simulink model "sm_car"  (R2025a)
settings: Solver=ode23t  StartTime=0.0  StopTime=400  MaxStep=0.4  RelTol=1e-3  AbsTol=1e-3  EnableMultiTasking=on
PreLoadFcn:
  | % Due to usability issue in Repeating Sequence block
  | warning('off','Simulink:Masking:Invalid');
  | 
  | % Eliminate unnecessary warnings in inactive variants
  | % Warnings generated only if you click through inactive variant
  | warning('off','MATLAB:nonExistentField');
  | warning('off','Simulink:Parameters:BlkParamUndefined');
PostLoadFcn:
  | set_param([bdroot '/Vehicle'],'popup_trailer','Off')
  | warning('off','sm:sli:setup:compile:LocalSolverNotSupported')
  | %sm_car_config_maneuver(bdroot,'WOT Braking');
  | sm_car_config_vehicle(bdroot,'false');
  | sm_car_config_logging(bdroot);
InitFcn:
  | sm_car_config_camera;
  | Vehicle = sm_car_vehcfg_checkConfig(Vehicle);
  | sm_car_check_tire_model(bdroot);
StartFcn:
  | tic;
StopFcn:
  | Elapsed_Sim_Time = toc;
  | % disp(['Elapsed Sim Time = ' num2str(Elapsed_Sim_Time)]);
undefined symbols (not defined in the file): Axle1D, AxleIn, Camera, Control, Driver, Free, Init, Maneuver, Pedal, RaceFix, RaceSpin, Scene, ShaftL1, ShaftL2, ShaftR1, ShaftR2, Soft, Stiff, Visual, X, xy_data_car_side, Y, Z
libraries: sm_lib x1546, nesl_utility x528, fl_lib x480, SimscapeFluids_lib x61, sdl_lib x49, simulink x29, ee_lib x7, simulink_extras x6, Linkage_Systems x4, Tire_1x2x x4, AntiRollBar_Systems x2, Linkage_Decoupled x2
(part 8 of 79)

== system sm_car/Vehicle/Vehicle/Chassis/Body ==
  Body Geometry : Subsystem  Variant=on  VariantControlMode=label  VariantControl=Variant1  LabelModeActiveChoice=CAD_FSAE_Achilles  mask(Variants for Vehicle Body Geometry){BodyGeometry=BodyGeometry, VariantLabel=BodyGeometry.class.Value}
      mask prompts: VariantLabel "Variant Label"
      mask help: Select option and provide parameters for vehicle body geometry. Option is chosen by string provided in Variant Label. The parameters for the selected option is contained in Body Geometry data structure.
      mask init:
      | curblk = gcb;
      | 
      | % Set variant for this block 
      | set_param(curblk,'LabelModeActiveChoice',VariantLabel);
      settings: AttributesFormatString=%<LabelModeActiveChoice>
  Body Load : Subsystem  Variant=on  VariantControlMode=label  VariantControl=Variant1  LabelModeActiveChoice=None  mask(Variants for Vehicle Body Load){BodyLoad=BodyLoad, VariantLabel=BodyLoad.class.Value}
      mask prompts: VariantLabel "Variant Label"
      mask help: Select option and provide parameters for vehicle body load. Option is chosen by string provided in Variant Label. The parameters for the selected option is contained in Body Load data structure.
      mask init:
      | curblk = gcb;
      | 
      | % Set variant for this block 
      | set_param(curblk,'LabelModeActiveChoice',VariantLabel);
      settings: AttributesFormatString=%<LabelModeActiveChoice>
  Body Mass and Inertia : sm_lib/Body Elements/Spherical Solid  SphereRadius=size_chassis_hp_cg  SphereRadiusUnits=m  ExportEntireGeometry=off  InertiaType=Custom  BasedOnType=Density  Density=312*0.6  DensityUnits=kg/m^3  Mass=chassis_mass  MassUnits=kg  CenterOfMass=[0 0 0]  CenterOfMassUnits=m  MomentsOfInertia=chassis_inertia  MomentsOfInertiaUnits=kg*m^2  ProductsOfInertia=[0 0 0]  ProductsOfInertiaUnits=kg*m^2  GraphicType=FromGeometry  MarkerShape=Sphere  MarkerSize=10  GraphicVisPropType=SimpleVisualProperties  GraphicDiffuseColor=clr_chassis_hp_cg  GraphicOpacity=opc_chassis_hp_cg  GraphicSpecularColor=[0.5 0.5 0.5 1.0]  GraphicAmbientColor=[0.15 0.15 0.15 1.0]  GraphicEmissiveColor=[0.0 0.0 0.0 1.0]  GraphicShininess=75  DoExposeReferenceFrame=on  SerializedFrames=<Frames/>
  Body Sensor : Subsystem  mask{offset_body_sensor=[0 0 0]}
      mask prompts: offset_body_sensor "Sensor Frame Offset [x y z] (m)"
  Bus Creator : BusCreator  Inputs=4
  Passenger FL : Subsystem  Variant=on  VariantControlMode=label  LabelModeActiveChoice=None  mask{Passenger=Passenger.FL, VariantLabel=Passenger.FL.class.Value}
      mask prompts: Passenger "Passenger Data"; VariantLabel "Variant Label"
      mask init:
      | curblk = gcb;
      | 
      | % Set variant for this block 
      | set_param(curblk,'LabelModeActiveChoice',VariantLabel);
      settings: AttributesFormatString=%<LabelModeActiveChoice>
  Passenger FR : Subsystem  Variant=on  VariantControlMode=label  LabelModeActiveChoice=None  mask{Passenger=Passenger.FR, VariantLabel=Passenger.FR.class.Value}
      mask prompts: Passenger "Passenger Data"; VariantLabel "Variant Label"
      mask init:
      | curblk = gcb;
      | 
      | % Set variant for this block 
      | set_param(curblk,'LabelModeActiveChoice',VariantLabel);
      settings: AttributesFormatString=%<LabelModeActiveChoice>
  Passenger RL : Subsystem  Variant=on  VariantControlMode=label  LabelModeActiveChoice=None  mask{Passenger=Passenger.RL, VariantLabel=Passenger.RL.class.Value}
      mask prompts: Passenger "Passenger Data"; VariantLabel "Variant Label"
      mask init:
      | curblk = gcb;
      | 
      | % Set variant for this block 
      | set_param(curblk,'LabelModeActiveChoice',VariantLabel);
      settings: AttributesFormatString=%<LabelModeActiveChoice>
  Passenger RR : Subsystem  Variant=on  VariantControlMode=label  LabelModeActiveChoice=None  mask{Passenger=Passenger.RR, VariantLabel=Passenger.RR.class.Value}
      mask prompts: Passenger "Passenger Data"; VariantLabel "Variant Label"
      mask init:
      | curblk = gcb;
      | 
      | % Set variant for this block 
      | set_param(curblk,'LabelModeActiveChoice',VariantLabel);
      settings: AttributesFormatString=%<LabelModeActiveChoice>
  Reference Frame Front Hitch : sm_lib/Frames and Transforms/Reference Frame
  Reference Frame Rear Hitch : sm_lib/Frames and Transforms/Reference Frame
  Transform Body CG : sm_lib/Frames and Transforms/Rigid Transform  RotationMethod=None  FollAlignAxisA=+X  BaseAlignAxisA=+Y  FollAlignAxisB=+Y  BaseAlignAxisB=+Z  RotationStandardAxis=+Z  RotationAngle=0.0  RotationAngleUnits=deg  RotationArbitraryAxis=[0 0 1]  RotationSequenceAxes=FollowerAxes  RotationSequence=XYX  RotationSequenceAngles=[0 0 0]  RotationSequenceAnglesUnits=deg  RotationMatrix=[1 0 0; 0 1 0; 0 0 1]  Quaternion=[1 0 0 0]  TranslationMethod=Cartesian  TranslationCartesianOffset=hp_chassis_cg  TranslationCartesianOffsetUnits=m  TranslationStandardAxis=+Z  TranslationStandardOffset=0  TranslationStandardOffsetUnits=m  TranslationROffset=0  TranslationROffsetUnits=m  TranslationThetaOffset=0  TranslationThetaOffsetUnits=deg  TranslationZOffset=0  TranslationZOffsetUnits=m
  Transform Front Hitch : sm_lib/Frames and Transforms/Rigid Transform  RotationMethod=None  FollAlignAxisA=+X  BaseAlignAxisA=+Y  FollAlignAxisB=+Y  BaseAlignAxisB=+Z  RotationStandardAxis=+Z  RotationAngle=0.0  RotationAngleUnits=deg  RotationArbitraryAxis=[0 0 1]  RotationSequenceAxes=FollowerAxes  RotationSequence=XYX  RotationSequenceAngles=[0 0 0]  RotationSequenceAnglesUnits=deg  RotationMatrix=[1 0 0; 0 1 0; 0 0 1]  Quaternion=[1 0 0 0]  TranslationMethod=Cartesian  TranslationCartesianOffset=hp_mount_hitchf  TranslationCartesianOffsetUnits=m  TranslationStandardAxis=-X  TranslationStandardOffset=0  TranslationStandardOffsetUnits=m  TranslationROffset=0  TranslationROffsetUnits=m  TranslationThetaOffset=0  TranslationThetaOffsetUnits=deg  TranslationZOffset=0  TranslationZOffsetUnits=m
  Transform Mount A1 : sm_lib/Frames and Transforms/Rigid Transform  RotationMethod=None  FollAlignAxisA=+X  BaseAlignAxisA=+Y  FollAlignAxisB=+Y  BaseAlignAxisB=+Z  RotationStandardAxis=+Z  RotationAngle=0.0  RotationAngleUnits=deg  RotationArbitraryAxis=[0 0 1]  RotationSequenceAxes=FollowerAxes  RotationSequence=XYX  RotationSequenceAngles=[0 0 0]  RotationSequenceAnglesUnits=deg  RotationMatrix=[1 0 0; 0 1 0; 0 0 1]  Quaternion=[1 0 0 0]  TranslationMethod=Cartesian  TranslationCartesianOffset=hp_mount_a1  TranslationCartesianOffsetUnits=m  TranslationStandardAxis=+X  TranslationStandardOffset=0  TranslationStandardOffsetUnits=m  TranslationROffset=0  TranslationROffsetUnits=m  TranslationThetaOffset=0  TranslationThetaOffsetUnits=deg  TranslationZOffset=0  TranslationZOffsetUnits=m
  Transform Mount A2 : sm_lib/Frames and Transforms/Rigid Transform  RotationMethod=None  FollAlignAxisA=+X  BaseAlignAxisA=+Y  FollAlignAxisB=+Y  BaseAlignAxisB=+Z  RotationStandardAxis=+Z  RotationAngle=0.0  RotationAngleUnits=deg  RotationArbitraryAxis=[0 0 1]  RotationSequenceAxes=FollowerAxes  RotationSequence=XYX  RotationSequenceAngles=[0 0 0]  RotationSequenceAnglesUnits=deg  RotationMatrix=[1 0 0; 0 1 0; 0 0 1]  Quaternion=[1 0 0 0]  TranslationMethod=Cartesian  TranslationCartesianOffset=hp_mount_a2  TranslationCartesianOffsetUnits=m  TranslationStandardAxis=-X  TranslationStandardOffset=0  TranslationStandardOffsetUnits=m  TranslationROffset=0  TranslationROffsetUnits=m  TranslationThetaOffset=0  TranslationThetaOffsetUnits=deg  TranslationZOffset=0  TranslationZOffsetUnits=m
  Transform Power Mount : sm_lib/Frames and Transforms/Rigid Transform  RotationMethod=None  FollAlignAxisA=+X  BaseAlignAxisA=+Y  FollAlignAxisB=+Y  BaseAlignAxisB=+Z  RotationStandardAxis=+Z  RotationAngle=0.0  RotationAngleUnits=deg  RotationArbitraryAxis=[0 0 1]  RotationSequenceAxes=FollowerAxes  RotationSequence=XYX  RotationSequenceAngles=[0 0 0]  RotationSequenceAnglesUnits=deg  RotationMatrix=[1 0 0; 0 1 0; 0 0 1]  Quaternion=[1 0 0 0]  TranslationMethod=Cartesian  TranslationCartesianOffset=hp_mount_power  TranslationCartesianOffsetUnits=m  TranslationStandardAxis=+Z  TranslationStandardOffset=0  TranslationStandardOffsetUnits=m  TranslationROffset=0  TranslationROffsetUnits=m  TranslationThetaOffset=0  TranslationThetaOffsetUnits=deg  TranslationZOffset=0  TranslationZOffsetUnits=m
  Transform Rear Hitch : sm_lib/Frames and Transforms/Rigid Transform  RotationMethod=None  FollAlignAxisA=+X  BaseAlignAxisA=+Y  FollAlignAxisB=+Y  BaseAlignAxisB=+Z  RotationStandardAxis=+Z  RotationAngle=0.0  RotationAngleUnits=deg  RotationArbitraryAxis=[0 0 1]  RotationSequenceAxes=FollowerAxes  RotationSequence=XYX  RotationSequenceAngles=[0 0 0]  RotationSequenceAnglesUnits=deg  RotationMatrix=[1 0 0; 0 1 0; 0 0 1]  Quaternion=[1 0 0 0]  TranslationMethod=Cartesian  TranslationCartesianOffset=hp_mount_hitchr  TranslationCartesianOffsetUnits=m  TranslationStandardAxis=-X  TranslationStandardOffset=0  TranslationStandardOffsetUnits=m  TranslationROffset=0  TranslationROffsetUnits=m  TranslationThetaOffset=0  TranslationThetaOffsetUnits=deg  TranslationZOffset=0  TranslationZOffsetUnits=m
  Vis HP Mount A1 : sm_lib/Body Elements/Spherical Solid  SphereRadius=size_chassis_hp_cg  SphereRadiusUnits=m  ExportEntireGeometry=off  InertiaType=PointMass  BasedOnType=Density  Density=312*0.6  DensityUnits=kg/m^3  Mass=0  MassUnits=kg  CenterOfMass=[0 0 0]  CenterOfMassUnits=m  MomentsOfInertia=[1 1 1]  MomentsOfInertiaUnits=kg*m^2  ProductsOfInertia=[0 0 0]  ProductsOfInertiaUnits=kg*m^2  GraphicType=FromGeometry  MarkerShape=Sphere  MarkerSize=10  GraphicVisPropType=SimpleVisualProperties  GraphicDiffuseColor=clr_chassis_hp_cg  GraphicOpacity=opc_chassis_hp_cg  GraphicSpecularColor=[0.5 0.5 0.5 1.0]  GraphicAmbientColor=[0.15 0.15 0.15 1.0]  GraphicEmissiveColor=[0.0 0.0 0.0 1.0]  GraphicShininess=75  DoExposeReferenceFrame=on  SerializedFrames=<Frames/>
  Vis HP Mount A2 : sm_lib/Body Elements/Spherical Solid  SphereRadius=size_chassis_hp_cg  SphereRadiusUnits=m  ExportEntireGeometry=off  InertiaType=PointMass  BasedOnType=Density  Density=312*0.6  DensityUnits=kg/m^3  Mass=0  MassUnits=kg  CenterOfMass=[0 0 0]  CenterOfMassUnits=m  MomentsOfInertia=[1 1 1]  MomentsOfInertiaUnits=kg*m^2  ProductsOfInertia=[0 0 0]  ProductsOfInertiaUnits=kg*m^2  GraphicType=FromGeometry  MarkerShape=Sphere  MarkerSize=10  GraphicVisPropType=SimpleVisualProperties  GraphicDiffuseColor=clr_chassis_hp_cg  GraphicOpacity=opc_chassis_hp_cg  GraphicSpecularColor=[0.5 0.5 0.5 1.0]  GraphicAmbientColor=[0.15 0.15 0.15 1.0]  GraphicEmissiveColor=[0.0 0.0 0.0 1.0]  GraphicShininess=75  DoExposeReferenceFrame=on  SerializedFrames=<Frames/>
  HF : PMIOPort  Side=Left
  A1 : PMIOPort  Port=2  Side=Right
  Pwr : PMIOPort  Port=3  Side=Left
  W : PMIOPort  Port=4  Side=Left
  A2 : PMIOPort  Port=5  Side=Right
  HR : PMIOPort  Port=6  Side=Left
  Out Bus Element : Outport  VectorParamsAs1DForOutWhenUnconnected=off  PortName=m  Element=Passengers
  Out Bus Element1 : Outport  VectorParamsAs1DForOutWhenUnconnected=off  PortName=m  Element=CG
  wires:
  Body Sensor/1(Body) -> Out Bus Element1/1
  [PassRR] -> Bus Creator/4  "RR"
  [PassRL] -> Bus Creator/3  "RL"
  Passenger RR/1(m) -> [PassRR]
  Passenger RL/1(m) -> [PassRL]
  Passenger FL/1(m) -> [PassFL]
  [PassFR] -> Bus Creator/2  "FR"
  [PassFL] -> Bus Creator/1  "FL"
  Passenger FR/1(m) -> [PassFR]
  Bus Creator/1 -> Out Bus Element/1
  connections:
  Passenger RR/LConn1 -- Passenger FR/LConn1 -- Passenger FL/LConn1 -- Body Geometry/LConn1 -- Passenger RL/LConn1
  Reference Frame Front Hitch/RConn1 -- Transform Front Hitch/RConn1 -- HF/RConn1
  Reference Frame Rear Hitch/RConn1 -- Transform Rear Hitch/RConn1 -- HR/RConn1
  Pwr/RConn1 -- Transform Power Mount/RConn1
  Transform Mount A2/RConn1 -- Vis HP Mount A2/RConn1 -- A2/RConn1
  Transform Mount A1/RConn1 -- Body Load/LConn1 -- Body Geometry/RConn1 -- A1/RConn1 -- Vis HP Mount A1/RConn1
  Transform Body CG/RConn1 -- Body Sensor/LConn1 -- Body Mass and Inertia/RConn1
  W/RConn1 -- Transform Rear Hitch/LConn1 -- Transform Front Hitch/LConn1 -- Transform Mount A1/LConn1 -- Transform Mount A2/LConn1 -- Transform Power Mount/LConn1 -- Transform Body CG/LConn1

== system sm_car/Vehicle/Vehicle/Chassis/Damper ==
  "Ctrl " : Inport
  Decoupled : Subsystem  VariantControl=Decoupled  mask(Roll and Heave Dampers){}
      mask help: Models dampers in a suspension design that decouples damping for body roll and heave .
  Independent : Subsystem  VariantControl=Independent  mask(Independent Dampers){}
      mask help: Models independent left and right dampers on two axles
  " L1" : PMIOPort  Side=Left
  " R1" : PMIOPort  Port=2  Side=Right
  " L2" : PMIOPort  Port=3  Side=Left
  " R2" : PMIOPort  Port=4  Side=Right
  " meas" : Outport  VectorParamsAs1DForOutWhenUnconnected=off

== system sm_car/Vehicle/Vehicle/Chassis/Spring ==
  "Ctrl " : Inport
  Decoupled : Subsystem  VariantControl=Decoupled  mask(Roll and Heave Springs){}
      mask help: Models springs in a suspension design that decouples stiffness for body roll and heave .
  Independent : Subsystem  VariantControl=Independent  mask(Independent Springs){}
      mask help: Models independent left and right springs on two axles
  " L1" : PMIOPort  Side=Left
  R1 : PMIOPort  Port=2  Side=Right
  " L2" : PMIOPort  Port=3  Side=Left
  R2 : PMIOPort  Port=4  Side=Right
  " meas" : Outport  VectorParamsAs1DForOutWhenUnconnected=off

== system sm_car/Vehicle/Vehicle/Chassis/SuspA1 ==
  "CtrlBus " : Inport
  DrvBus : Inport  Port=2
  Linkage : Subsystem  VariantControl=Linkage  mask(Linkage Suspension){}
      mask help: Models suspension using linkages, including double-wishbone and multi-link suspensions. This subsystem models the suspension, spring and damper parts, and optional steering system. The displacement of the springs and dampers are modeled here and the forces are modeled in a separate subsystem.
      mask Display: image('sm_car_vehicle_susp_linkage_IMAGE.png');
  Linkage Decoupled : Subsystem  VariantControl=Decoupled  mask(Linkage Decoupled){}
      mask help: Models suspension using a linkage where the stiffness and damping for the roll and heave degrees of freedom are decoupled. Includes suspension, spring and damper parts, and optional steering system. The displacement of the springs and dampers are modeled here and the forces are modeled in a separate subsystem.
      mask Display: image('sm_car_vehicle_susp_linkage_decouple_IMAGE.png');
  WCL : PMIOPort  Side=Left
  Ref : PMIOPort  Port=2  Side=Right
  WCR : PMIOPort  Port=3  Side=Right
  AxleL : PMIOPort  Port=4  Side=Left
  AxleR : PMIOPort  Port=5  Side=Right
  SprL : PMIOPort  Port=6  Side=Left
  SprR : PMIOPort  Port=7  Side=Right
  DmpL : PMIOPort  Port=8  Side=Left
  DmpR : PMIOPort  Port=9  Side=Right
  OutBus : Outport  VectorParamsAs1DForOutWhenUnconnected=off

== system sm_car/Vehicle/Vehicle/Chassis/SuspA2 ==
  "CtrlBus " : Inport
  DrvBus : Inport  Port=2
  Linkage : Subsystem  VariantControl=Linkage  mask(Linkage Suspension){}
      mask help: Models suspension using linkages, including double-wishbone and multi-link suspensions. This subsystem models the suspension, spring and damper parts, and optional steering system. The displacement of the springs and dampers are modeled here and the forces are modeled in a separate subsystem.
      mask Display: image('sm_car_vehicle_susp_linkage_IMAGE.png');
  Linkage Decoupled : Suspension_Linkage_Decoupled/Linkage Decoupled  VariantControl=Decoupled
  WCL : PMIOPort  Side=Left
  Ref : PMIOPort  Port=2  Side=Right
  WCR : PMIOPort  Port=3  Side=Right
  AxleL : PMIOPort  Port=4  Side=Left
  AxleR : PMIOPort  Port=5  Side=Right
  SprL : PMIOPort  Port=6  Side=Left
  SprR : PMIOPort  Port=7  Side=Right
  DmpL : PMIOPort  Port=8  Side=Left
  DmpR : PMIOPort  Port=9  Side=Right
  OutBus : Outport  VectorParamsAs1DForOutWhenUnconnected=off

== system sm_car/Vehicle/Vehicle/Powertrain/Driveline ==
  CtrlBus : Inport
  L1 R1 L2 R2 : Subsystem  Tag=PublishSubsystem  VariantControl=L1_R1_L2_R2  mask(Driveline, Two-Axle, Four Input Shaft){}
      mask help: Models two-axle driveline with four separate shafts. The shafts are connected independently to the wheels.
      mask Display: image('sm_car_vehicle_driveline_axle2_l1_r1_l2_r2_IMAGE.png');
  A1 : PMIOPort  Side=Left
  A2 : PMIOPort  Port=2  Side=Right
  L1 : PMIOPort  Port=3  Side=Left
  R1 : PMIOPort  Port=4  Side=Right
  L2 : PMIOPort  Port=5  Side=Left
  R2 : PMIOPort  Port=6  Side=Right
  Shafts : PMIOPort  Port=7  Side=Left
  " o" : PMIOPort  Port=8  Side=Right
  OutD : Outport  VectorParamsAs1DForOutWhenUnconnected=off

== system sm_car/Vehicle/Vehicle/Powertrain/Power ==
  CtrlBus : Inport
  VehBus : Inport  Port=2
  Electric L1 R1 L2 R2 : Subsystem  VariantControl=Electric_L1_R1_L2_R2  mask(Electric Propulsion with Four Motors){Power=Powertrain.Power}
      mask prompts: Power "Power 4 Motor (structure)"
      mask help: Four electric motors with optional cooling system. Physical connections for the four motor shafts are in bus Shafts.
      mask Display: image('sm_car_vehicle_power_e4motor_IMAGE.png');
  Shafts : PMIOPort  Side=Left
  Ref : PMIOPort  Port=2  Side=Right
  OutP : Outport  VectorParamsAs1DForOutWhenUnconnected=off

== system sm_car/Vehicle/Vehicle/Wheel Spin/Free ==
  note: For kinematics and compliance tests, the wheels need to be locked so they cannot spin.
      |
      | For all other tests, they should be free to rotate.
  L1 : PMIOPort  Side=Left
  L2 : PMIOPort  Port=2  Side=Left
  R1 : PMIOPort  Port=3  Side=Right
  R2 : PMIOPort  Port=4  Side=Right

== system sm_car/World/Scene/CRG Hockenheim/Finish Line ==
  L1 : Subsystem  mask{square_lwh=[0.01 1 1]}
      mask prompts: square_lwh "Size [l w h] (m)"
  L2 : Subsystem  mask{square_lwh=[0.01 1 1]}
      mask prompts: square_lwh "Size [l w h] (m)"
  L3 : Subsystem  mask{square_lwh=[0.01 1 1]}
      mask prompts: square_lwh "Size [l w h] (m)"
  L4 : Subsystem  mask{square_lwh=[0.01 1 1]}
      mask prompts: square_lwh "Size [l w h] (m)"
  L5 : Subsystem  mask{square_lwh=[0.01 1 1]}
      mask prompts: square_lwh "Size [l w h] (m)"
  Post L : sm_lib/Body Elements/Cylindrical Solid  CylinderRadius=post_r  CylinderRadiusUnits=m  CylinderLength=post_h  CylinderLengthUnits=m  ExportEntireGeometry=off  InertiaType=CalculateFromGeometry  BasedOnType=Density  Density=1000  DensityUnits=kg/m^3  Mass=1  MassUnits=kg  CenterOfMass=[0 0 0]  CenterOfMassUnits=m  MomentsOfInertia=[1 1 1]  MomentsOfInertiaUnits=kg*m^2  ProductsOfInertia=[0 0 0]  ProductsOfInertiaUnits=kg*m^2  GraphicType=FromGeometry  MarkerShape=Sphere  MarkerSize=10  GraphicVisPropType=SimpleVisualProperties  GraphicDiffuseColor=post_clr  GraphicOpacity=post_opc  GraphicSpecularColor=[0.5 0.5 0.5 1.0]  GraphicAmbientColor=[0.15 0.15 0.15 1.0]  GraphicEmissiveColor=[0.0 0.0 0.0 1.0]  GraphicShininess=75  DoExposeReferenceFrame=off  SerializedFrames=<Frames><Frame><Id>Frame1</Id><Value><Name>B</Name><Origin><Source>GeometricFeature</Source><FeatureName>bottom surface</FeatureName></Origin><PrimaryAxis><DefinedDirection>+Z</DefinedDirection><Source>ReferenceFrame</Source><SourceDirection>+Z</SourceDirection><FeatureName></FeatureName></PrimaryAxis><SecondaryAxis><DefinedDirection>+X</DefinedDirection><Source>ReferenceFrame</Source><SourceDirection>+X</SourceDirection><FeatureName></FeatureName></SecondaryAxis></Value></Frame><Frame><Id>Frame2</Id><Value><Name>T</Name><Origin><Source>GeometricFeature</Source><FeatureName>top surface</FeatureName></Origin><PrimaryAxis><DefinedDirection>+Z</DefinedDirection><Source>ReferenceFrame</Source><SourceDirection>+Z</SourceDirection><FeatureName></FeatureName></PrimaryAxis><SecondaryAxis><DefinedDirection>+X</DefinedDirection><Source>ReferenceFrame</Source><SourceDirection>+X</SourceDirection><FeatureName></FeatureName></SecondaryAxis></Value></Frame></Frames>
  Post R : sm_lib/Body Elements/Cylindrical Solid  CylinderRadius=post_r  CylinderRadiusUnits=m  CylinderLength=post_h  CylinderLengthUnits=m  ExportEntireGeometry=off  InertiaType=CalculateFromGeometry  BasedOnType=Density  Density=1000  DensityUnits=kg/m^3  Mass=1  MassUnits=kg  CenterOfMass=[0 0 0]  CenterOfMassUnits=m  MomentsOfInertia=[1 1 1]  MomentsOfInertiaUnits=kg*m^2  ProductsOfInertia=[0 0 0]  ProductsOfInertiaUnits=kg*m^2  GraphicType=FromGeometry  MarkerShape=Sphere  MarkerSize=10  GraphicVisPropType=SimpleVisualProperties  GraphicDiffuseColor=post_clr  GraphicOpacity=post_opc  GraphicSpecularColor=[0.5 0.5 0.5 1.0]  GraphicAmbientColor=[0.15 0.15 0.15 1.0]  GraphicEmissiveColor=[0.0 0.0 0.0 1.0]  GraphicShininess=75  DoExposeReferenceFrame=off  SerializedFrames=<Frames><Frame><Id>Frame1</Id><Value><Name>B</Name><Origin><Source>GeometricFeature</Source><FeatureName>bottom surface</FeatureName></Origin><PrimaryAxis><DefinedDirection>+Z</DefinedDirection><Source>ReferenceFrame</Source><SourceDirection>+Z</SourceDirection><FeatureName></FeatureName></PrimaryAxis><SecondaryAxis><DefinedDirection>+X</DefinedDirection><Source>ReferenceFrame</Source><SourceDirection>+X</SourceDirection><FeatureName></FeatureName></SecondaryAxis></Value></Frame><Frame><Id>Frame2</Id><Value><Name>T</Name><Origin><Source>GeometricFeature</Source><FeatureName>top surface</FeatureName></Origin><PrimaryAxis><DefinedDirection>+Z</DefinedDirection><Source>ReferenceFrame</Source><SourceDirection>+Z</SourceDirection><FeatureName></FeatureName></PrimaryAxis><SecondaryAxis><DefinedDirection>+X</DefinedDirection><Source>ReferenceFrame</Source><SourceDirection>+X</SourceDirection><FeatureName></FeatureName></SecondaryAxis></Value></Frame></Frames>
  R1 : Subsystem  mask{square_lwh=[0.01 1 1]}
      mask prompts: square_lwh "Size [l w h] (m)"
  R2 : Subsystem  mask{square_lwh=[0.01 1 1]}
      mask prompts: square_lwh "Size [l w h] (m)"
  R3 : Subsystem  mask{square_lwh=[0.01 1 1]}
      mask prompts: square_lwh "Size [l w h] (m)"
  R4 : Subsystem  mask{square_lwh=[0.01 1 1]}
      mask prompts: square_lwh "Size [l w h] (m)"
  R5 : Subsystem  mask{square_lwh=[0.01 1 1]}
      mask prompts: square_lwh "Size [l w h] (m)"
  Transform Orient Line : sm_lib/Frames and Transforms/Rigid Transform  RotationMethod=RotationSequence  FollAlignAxisA=+X  BaseAlignAxisA=+Y  FollAlignAxisB=+Y  BaseAlignAxisB=+Z  RotationStandardAxis=+Z  RotationAngle=0  RotationAngleUnits=deg  RotationArbitraryAxis=[0 0 1]  RotationSequenceAxes=FollowerAxes  RotationSequence=ZYX  RotationSequenceAngles=[offset_yaw offset_pitch offset_roll]  RotationSequenceAnglesUnits=rad  RotationMatrix=[1 0 0; 0 1 0; 0 0 1]  Quaternion=[1 0 0 0]  TranslationMethod=Cartesian  TranslationCartesianOffset=offset_xyz  TranslationCartesianOffsetUnits=m  TranslationStandardAxis=+Z  TranslationStandardOffset=0  TranslationStandardOffsetUnits=m  TranslationROffset=0  TranslationROffsetUnits=m  TranslationThetaOffset=0  TranslationThetaOffsetUnits=deg  TranslationZOffset=0  TranslationZOffsetUnits=m
  Transform Post L : sm_lib/Frames and Transforms/Rigid Transform  RotationMethod=StandardAxis  FollAlignAxisA=+X  BaseAlignAxisA=+Y  FollAlignAxisB=+Y  BaseAlignAxisB=+Z  RotationStandardAxis=+Y  RotationAngle=0.0  RotationAngleUnits=deg  RotationArbitraryAxis=[0 0 1]  RotationSequenceAxes=FollowerAxes  RotationSequence=XYX  RotationSequenceAngles=[0 0 0]  RotationSequenceAnglesUnits=deg  RotationMatrix=[1 0 0; 0 1 0; 0 0 1]  Quaternion=[1 0 0 0]  TranslationMethod=StandardAxis  TranslationCartesianOffset=[0 0 0]  TranslationCartesianOffsetUnits=m  TranslationStandardAxis=+Y  TranslationStandardOffset=line_w/2  TranslationStandardOffsetUnits=m  TranslationROffset=0  TranslationROffsetUnits=m  TranslationThetaOffset=0  TranslationThetaOffsetUnits=deg  TranslationZOffset=0  TranslationZOffsetUnits=m
  Transform Post R : sm_lib/Frames and Transforms/Rigid Transform  RotationMethod=StandardAxis  FollAlignAxisA=+X  BaseAlignAxisA=+Y  FollAlignAxisB=+Y  BaseAlignAxisB=+Z  RotationStandardAxis=+Y  RotationAngle=0.0  RotationAngleUnits=deg  RotationArbitraryAxis=[0 0 1]  RotationSequenceAxes=FollowerAxes  RotationSequence=XYX  RotationSequenceAngles=[0 0 0]  RotationSequenceAnglesUnits=deg  RotationMatrix=[1 0 0; 0 1 0; 0 0 1]  Quaternion=[1 0 0 0]  TranslationMethod=StandardAxis  TranslationCartesianOffset=[0 0 0]  TranslationCartesianOffsetUnits=m  TranslationStandardAxis=+Y  TranslationStandardOffset=line_w/2  TranslationStandardOffsetUnits=m  TranslationROffset=0  TranslationROffsetUnits=m  TranslationThetaOffset=0  TranslationThetaOffsetUnits=deg  TranslationZOffset=0  TranslationZOffsetUnits=m
  W : PMIOPort  Side=Left
  connections:
  Post R/RConn1 -- R1/RConn1
  R2/RConn1 -- R1/LConn1
  L2/RConn1 -- L3/LConn1
  R4/RConn1 -- R3/LConn1
  Transform Post R/LConn1 -- Post R/LConn1
  L3/RConn1 -- L4/LConn1
  Post L/LConn1 -- Transform Post L/RConn1
  W/RConn1 -- Transform Orient Line/LConn1
  R2/LConn1 -- R3/RConn1
  L5/LConn1 -- L4/RConn1
  R5/RConn1 -- R4/LConn1
  L1/RConn1 -- L2/LConn1
  L1/LConn1 -- Post L/RConn1
  Transform Post L/LConn1 -- Transform Orient Line/RConn1 -- Transform Post R/RConn1

== system sm_car/World/Scene/CRG Hockenheim/STL Geometry Centerline ==
  Geometry : sm_lib/Body Elements/File Solid  ExtGeomFileName=CRG_Hockenheim_centerline.stl  UnitType=Custom  ExtGeomFileUnits=m  StepReaderType=HEX  ExportConvexHullGeometry=off  InertiaType=Custom  BasedOnType=DensityFromFile  Density=1000  DensityUnits=kg/m^3  Mass=1  MassUnits=kg  CenterOfMass=[0 0 0]  CenterOfMassUnits=m  MomentsOfInertia=[1 1 1]  MomentsOfInertiaUnits=kg*m^2  ProductsOfInertia=[0 0 0]  ProductsOfInertiaUnits=kg*m^2  GraphicType=FromGeometry  MarkerShape=Sphere  MarkerSize=10  GraphicVisPropType=SimpleVisualProperties  GraphicDiffuseColor=stl_clr  GraphicOpacity=stl_opc  GraphicSpecularColor=[0.5 0.5 0.5 1.0]  GraphicAmbientColor=[0.15 0.15 0.15 1.0]  GraphicEmissiveColor=[0.0 0.0 0.0 1.0]  GraphicShininess=75  DoExposeReferenceFrame=on  SerializedFrames=<Frames/>
  Transform Geometry : sm_lib/Frames and Transforms/Rigid Transform  RotationMethod=RotationSequence  FollAlignAxisA=+X  BaseAlignAxisA=+Y  FollAlignAxisB=+Y  BaseAlignAxisB=+Z  RotationStandardAxis=+Z  RotationAngle=0  RotationAngleUnits=rad  RotationArbitraryAxis=[0 0 1]  RotationSequenceAxes=FollowerAxes  RotationSequence=ZYX  RotationSequenceAngles=[stl_yaw stl_pitch stl_roll]  RotationSequenceAnglesUnits=rad  RotationMatrix=[1 0 0; 0 1 0; 0 0 1]  Quaternion=[1 0 0 0]  TranslationMethod=Cartesian  TranslationCartesianOffset=[stl_x stl_y stl_z]  TranslationCartesianOffsetUnits=m  TranslationStandardAxis=+Z  TranslationStandardOffset=0  TranslationStandardOffsetUnits=m  TranslationROffset=0  TranslationROffsetUnits=m  TranslationThetaOffset=0  TranslationThetaOffsetUnits=deg  TranslationZOffset=0  TranslationZOffsetUnits=m
  W : PMIOPort  Side=Right
  connections:
  Geometry/RConn1 -- Transform Geometry/RConn1
  Transform Geometry/LConn1 -- W/RConn1

== system sm_car/World/Scene/CRG Hockenheim/STL Geometry Road ==
  Geometry : sm_lib/Body Elements/File Solid  ExtGeomFileName=CRG_Hockenheim.stl  UnitType=Custom  ExtGeomFileUnits=m  StepReaderType=HEX  ExportConvexHullGeometry=off  InertiaType=Custom  BasedOnType=DensityFromFile  Density=1000  DensityUnits=kg/m^3  Mass=1  MassUnits=kg  CenterOfMass=[0 0 0]  CenterOfMassUnits=m  MomentsOfInertia=[1 1 1]  MomentsOfInertiaUnits=kg*m^2  ProductsOfInertia=[0 0 0]  ProductsOfInertiaUnits=kg*m^2  GraphicType=FromGeometry  MarkerShape=Sphere  MarkerSize=10  GraphicVisPropType=SimpleVisualProperties  GraphicDiffuseColor=stl_clr  GraphicOpacity=stl_opc  GraphicSpecularColor=[0.5 0.5 0.5 1.0]  GraphicAmbientColor=[0.15 0.15 0.15 1.0]  GraphicEmissiveColor=[0.0 0.0 0.0 1.0]  GraphicShininess=75  DoExposeReferenceFrame=on  SerializedFrames=<Frames/>
  Transform Geometry : sm_lib/Frames and Transforms/Rigid Transform  RotationMethod=RotationSequence  FollAlignAxisA=+X  BaseAlignAxisA=+Y  FollAlignAxisB=+Y  BaseAlignAxisB=+Z  RotationStandardAxis=+Z  RotationAngle=0  RotationAngleUnits=rad  RotationArbitraryAxis=[0 0 1]  RotationSequenceAxes=FollowerAxes  RotationSequence=ZYX  RotationSequenceAngles=[stl_yaw stl_pitch stl_roll]  RotationSequenceAnglesUnits=rad  RotationMatrix=[1 0 0; 0 1 0; 0 0 1]  Quaternion=[1 0 0 0]  TranslationMethod=Cartesian  TranslationCartesianOffset=[stl_x stl_y stl_z]  TranslationCartesianOffsetUnits=m  TranslationStandardAxis=+Z  TranslationStandardOffset=0  TranslationStandardOffsetUnits=m  TranslationROffset=0  TranslationROffsetUnits=m  TranslationThetaOffset=0  TranslationThetaOffsetUnits=deg  TranslationZOffset=0  TranslationZOffsetUnits=m
  W : PMIOPort  Side=Right
  connections:
  Geometry/RConn1 -- Transform Geometry/RConn1
  Transform Geometry/LConn1 -- W/RConn1

== system sm_car/World/Scene/CRG Hockenheim F/Finish Line ==
  L1 : Subsystem  mask{square_lwh=[0.01 1 1]}
      mask prompts: square_lwh "Size [l w h] (m)"
  L2 : Subsystem  mask{square_lwh=[0.01 1 1]}
      mask prompts: square_lwh "Size [l w h] (m)"
  L3 : Subsystem  mask{square_lwh=[0.01 1 1]}
      mask prompts: square_lwh "Size [l w h] (m)"
  L4 : Subsystem  mask{square_lwh=[0.01 1 1]}
      mask prompts: square_lwh "Size [l w h] (m)"
  L5 : Subsystem  mask{square_lwh=[0.01 1 1]}
      mask prompts: square_lwh "Size [l w h] (m)"
  Post L : sm_lib/Body Elements/Cylindrical Solid  CylinderRadius=post_r  CylinderRadiusUnits=m  CylinderLength=post_h  CylinderLengthUnits=m  ExportEntireGeometry=off  InertiaType=CalculateFromGeometry  BasedOnType=Density  Density=1000  DensityUnits=kg/m^3  Mass=1  MassUnits=kg  CenterOfMass=[0 0 0]  CenterOfMassUnits=m  MomentsOfInertia=[1 1 1]  MomentsOfInertiaUnits=kg*m^2  ProductsOfInertia=[0 0 0]  ProductsOfInertiaUnits=kg*m^2  GraphicType=FromGeometry  MarkerShape=Sphere  MarkerSize=10  GraphicVisPropType=SimpleVisualProperties  GraphicDiffuseColor=post_clr  GraphicOpacity=post_opc  GraphicSpecularColor=[0.5 0.5 0.5 1.0]  GraphicAmbientColor=[0.15 0.15 0.15 1.0]  GraphicEmissiveColor=[0.0 0.0 0.0 1.0]  GraphicShininess=75  DoExposeReferenceFrame=off  SerializedFrames=<Frames><Frame><Id>Frame1</Id><Value><Name>B</Name><Origin><Source>GeometricFeature</Source><FeatureName>bottom surface</FeatureName></Origin><PrimaryAxis><DefinedDirection>+Z</DefinedDirection><Source>ReferenceFrame</Source><SourceDirection>+Z</SourceDirection><FeatureName></FeatureName></PrimaryAxis><SecondaryAxis><DefinedDirection>+X</DefinedDirection><Source>ReferenceFrame</Source><SourceDirection>+X</SourceDirection><FeatureName></FeatureName></SecondaryAxis></Value></Frame><Frame><Id>Frame2</Id><Value><Name>T</Name><Origin><Source>GeometricFeature</Source><FeatureName>top surface</FeatureName></Origin><PrimaryAxis><DefinedDirection>+Z</DefinedDirection><Source>ReferenceFrame</Source><SourceDirection>+Z</SourceDirection><FeatureName></FeatureName></PrimaryAxis><SecondaryAxis><DefinedDirection>+X</DefinedDirection><Source>ReferenceFrame</Source><SourceDirection>+X</SourceDirection><FeatureName></FeatureName></SecondaryAxis></Value></Frame></Frames>
  Post R : sm_lib/Body Elements/Cylindrical Solid  CylinderRadius=post_r  CylinderRadiusUnits=m  CylinderLength=post_h  CylinderLengthUnits=m  ExportEntireGeometry=off  InertiaType=CalculateFromGeometry  BasedOnType=Density  Density=1000  DensityUnits=kg/m^3  Mass=1  MassUnits=kg  CenterOfMass=[0 0 0]  CenterOfMassUnits=m  MomentsOfInertia=[1 1 1]  MomentsOfInertiaUnits=kg*m^2  ProductsOfInertia=[0 0 0]  ProductsOfInertiaUnits=kg*m^2  GraphicType=FromGeometry  MarkerShape=Sphere  MarkerSize=10  GraphicVisPropType=SimpleVisualProperties  GraphicDiffuseColor=post_clr  GraphicOpacity=post_opc  GraphicSpecularColor=[0.5 0.5 0.5 1.0]  GraphicAmbientColor=[0.15 0.15 0.15 1.0]  GraphicEmissiveColor=[0.0 0.0 0.0 1.0]  GraphicShininess=75  DoExposeReferenceFrame=off  SerializedFrames=<Frames><Frame><Id>Frame1</Id><Value><Name>B</Name><Origin><Source>GeometricFeature</Source><FeatureName>bottom surface</FeatureName></Origin><PrimaryAxis><DefinedDirection>+Z</DefinedDirection><Source>ReferenceFrame</Source><SourceDirection>+Z</SourceDirection><FeatureName></FeatureName></PrimaryAxis><SecondaryAxis><DefinedDirection>+X</DefinedDirection><Source>ReferenceFrame</Source><SourceDirection>+X</SourceDirection><FeatureName></FeatureName></SecondaryAxis></Value></Frame><Frame><Id>Frame2</Id><Value><Name>T</Name><Origin><Source>GeometricFeature</Source><FeatureName>top surface</FeatureName></Origin><PrimaryAxis><DefinedDirection>+Z</DefinedDirection><Source>ReferenceFrame</Source><SourceDirection>+Z</SourceDirection><FeatureName></FeatureName></PrimaryAxis><SecondaryAxis><DefinedDirection>+X</DefinedDirection><Source>ReferenceFrame</Source><SourceDirection>+X</SourceDirection><FeatureName></FeatureName></SecondaryAxis></Value></Frame></Frames>
  R1 : Subsystem  mask{square_lwh=[0.01 1 1]}
      mask prompts: square_lwh "Size [l w h] (m)"
  R2 : Subsystem  mask{square_lwh=[0.01 1 1]}
      mask prompts: square_lwh "Size [l w h] (m)"
  R3 : Subsystem  mask{square_lwh=[0.01 1 1]}
      mask prompts: square_lwh "Size [l w h] (m)"
  R4 : Subsystem  mask{square_lwh=[0.01 1 1]}
      mask prompts: square_lwh "Size [l w h] (m)"
  R5 : Subsystem  mask{square_lwh=[0.01 1 1]}
      mask prompts: square_lwh "Size [l w h] (m)"
  Transform Orient Line : sm_lib/Frames and Transforms/Rigid Transform  RotationMethod=RotationSequence  FollAlignAxisA=+X  BaseAlignAxisA=+Y  FollAlignAxisB=+Y  BaseAlignAxisB=+Z  RotationStandardAxis=+Z  RotationAngle=0  RotationAngleUnits=deg  RotationArbitraryAxis=[0 0 1]  RotationSequenceAxes=FollowerAxes  RotationSequence=ZYX  RotationSequenceAngles=[offset_yaw offset_pitch offset_roll]  RotationSequenceAnglesUnits=rad  RotationMatrix=[1 0 0; 0 1 0; 0 0 1]  Quaternion=[1 0 0 0]  TranslationMethod=Cartesian  TranslationCartesianOffset=offset_xyz  TranslationCartesianOffsetUnits=m  TranslationStandardAxis=+Z  TranslationStandardOffset=0  TranslationStandardOffsetUnits=m  TranslationROffset=0  TranslationROffsetUnits=m  TranslationThetaOffset=0  TranslationThetaOffsetUnits=deg  TranslationZOffset=0  TranslationZOffsetUnits=m
  Transform Post L : sm_lib/Frames and Transforms/Rigid Transform  RotationMethod=StandardAxis  FollAlignAxisA=+X  BaseAlignAxisA=+Y  FollAlignAxisB=+Y  BaseAlignAxisB=+Z  RotationStandardAxis=+Y  RotationAngle=0.0  RotationAngleUnits=deg  RotationArbitraryAxis=[0 0 1]  RotationSequenceAxes=FollowerAxes  RotationSequence=XYX  RotationSequenceAngles=[0 0 0]  RotationSequenceAnglesUnits=deg  RotationMatrix=[1 0 0; 0 1 0; 0 0 1]  Quaternion=[1 0 0 0]  TranslationMethod=StandardAxis  TranslationCartesianOffset=[0 0 0]  TranslationCartesianOffsetUnits=m  TranslationStandardAxis=+Y  TranslationStandardOffset=line_w/2  TranslationStandardOffsetUnits=m  TranslationROffset=0  TranslationROffsetUnits=m  TranslationThetaOffset=0  TranslationThetaOffsetUnits=deg  TranslationZOffset=0  TranslationZOffsetUnits=m
  Transform Post R : sm_lib/Frames and Transforms/Rigid Transform  RotationMethod=StandardAxis  FollAlignAxisA=+X  BaseAlignAxisA=+Y  FollAlignAxisB=+Y  BaseAlignAxisB=+Z  RotationStandardAxis=+Y  RotationAngle=0.0  RotationAngleUnits=deg  RotationArbitraryAxis=[0 0 1]  RotationSequenceAxes=FollowerAxes  RotationSequence=XYX  RotationSequenceAngles=[0 0 0]  RotationSequenceAnglesUnits=deg  RotationMatrix=[1 0 0; 0 1 0; 0 0 1]  Quaternion=[1 0 0 0]  TranslationMethod=StandardAxis  TranslationCartesianOffset=[0 0 0]  TranslationCartesianOffsetUnits=m  TranslationStandardAxis=+Y  TranslationStandardOffset=line_w/2  TranslationStandardOffsetUnits=m  TranslationROffset=0  TranslationROffsetUnits=m  TranslationThetaOffset=0  TranslationThetaOffsetUnits=deg  TranslationZOffset=0  TranslationZOffsetUnits=m
  W : PMIOPort  Side=Left
  connections:
  Post R/RConn1 -- R1/RConn1
  R2/RConn1 -- R1/LConn1
  L2/RConn1 -- L3/LConn1
  R4/RConn1 -- R3/LConn1
  Transform Post R/LConn1 -- Post R/LConn1
  L3/RConn1 -- L4/LConn1
  Post L/LConn1 -- Transform Post L/RConn1
  W/RConn1 -- Transform Orient Line/LConn1
  R2/LConn1 -- R3/RConn1
  L5/LConn1 -- L4/RConn1
  R5/RConn1 -- R4/LConn1
  L1/RConn1 -- L2/LConn1
  L1/LConn1 -- Post L/RConn1
  Transform Post L/LConn1 -- Transform Orient Line/RConn1 -- Transform Post R/RConn1

== system sm_car/World/Scene/CRG Hockenheim F/STL Geometry Centerline ==
  Geometry : sm_lib/Body Elements/File Solid  ExtGeomFileName=CRG_Hockenheim_f_centerline.stl  UnitType=Custom  ExtGeomFileUnits=m  StepReaderType=HEX  ExportConvexHullGeometry=off  InertiaType=Custom  BasedOnType=DensityFromFile  Density=1000  DensityUnits=kg/m^3  Mass=1  MassUnits=kg  CenterOfMass=[0 0 0]  CenterOfMassUnits=m  MomentsOfInertia=[1 1 1]  MomentsOfInertiaUnits=kg*m^2  ProductsOfInertia=[0 0 0]  ProductsOfInertiaUnits=kg*m^2  GraphicType=FromGeometry  MarkerShape=Sphere  MarkerSize=10  GraphicVisPropType=SimpleVisualProperties  GraphicDiffuseColor=stl_clr  GraphicOpacity=stl_opc  GraphicSpecularColor=[0.5 0.5 0.5 1.0]  GraphicAmbientColor=[0.15 0.15 0.15 1.0]  GraphicEmissiveColor=[0.0 0.0 0.0 1.0]  GraphicShininess=75  DoExposeReferenceFrame=on  SerializedFrames=<Frames/>
  Transform Geometry : sm_lib/Frames and Transforms/Rigid Transform  RotationMethod=RotationSequence  FollAlignAxisA=+X  BaseAlignAxisA=+Y  FollAlignAxisB=+Y  BaseAlignAxisB=+Z  RotationStandardAxis=+Z  RotationAngle=0  RotationAngleUnits=rad  RotationArbitraryAxis=[0 0 1]  RotationSequenceAxes=FollowerAxes  RotationSequence=ZYX  RotationSequenceAngles=[stl_yaw stl_pitch stl_roll]  RotationSequenceAnglesUnits=rad  RotationMatrix=[1 0 0; 0 1 0; 0 0 1]  Quaternion=[1 0 0 0]  TranslationMethod=Cartesian  TranslationCartesianOffset=[stl_x stl_y stl_z]  TranslationCartesianOffsetUnits=m  TranslationStandardAxis=+Z  TranslationStandardOffset=0  TranslationStandardOffsetUnits=m  TranslationROffset=0  TranslationROffsetUnits=m  TranslationThetaOffset=0  TranslationThetaOffsetUnits=deg  TranslationZOffset=0  TranslationZOffsetUnits=m
  W : PMIOPort  Side=Right
  connections:
  Geometry/RConn1 -- Transform Geometry/RConn1
  Transform Geometry/LConn1 -- W/RConn1

== system sm_car/World/Scene/CRG Hockenheim F/STL Geometry Road ==
  Geometry : sm_lib/Body Elements/File Solid  ExtGeomFileName=CRG_Hockenheim_f.stl  UnitType=Custom  ExtGeomFileUnits=m  StepReaderType=HEX  ExportConvexHullGeometry=off  InertiaType=Custom  BasedOnType=DensityFromFile  Density=1000  DensityUnits=kg/m^3  Mass=1  MassUnits=kg  CenterOfMass=[0 0 0]  CenterOfMassUnits=m  MomentsOfInertia=[1 1 1]  MomentsOfInertiaUnits=kg*m^2  ProductsOfInertia=[0 0 0]  ProductsOfInertiaUnits=kg*m^2  GraphicType=FromGeometry  MarkerShape=Sphere  MarkerSize=10  GraphicVisPropType=SimpleVisualProperties  GraphicDiffuseColor=stl_clr  GraphicOpacity=stl_opc  GraphicSpecularColor=[0.5 0.5 0.5 1.0]  GraphicAmbientColor=[0.15 0.15 0.15 1.0]  GraphicEmissiveColor=[0.0 0.0 0.0 1.0]  GraphicShininess=75  DoExposeReferenceFrame=on  SerializedFrames=<Frames/>
  Transform Geometry : sm_lib/Frames and Transforms/Rigid Transform  RotationMethod=RotationSequence  FollAlignAxisA=+X  BaseAlignAxisA=+Y  FollAlignAxisB=+Y  BaseAlignAxisB=+Z  RotationStandardAxis=+Z  RotationAngle=0  RotationAngleUnits=rad  RotationArbitraryAxis=[0 0 1]  RotationSequenceAxes=FollowerAxes  RotationSequence=ZYX  RotationSequenceAngles=[stl_yaw stl_pitch stl_roll]  RotationSequenceAnglesUnits=rad  RotationMatrix=[1 0 0; 0 1 0; 0 0 1]  Quaternion=[1 0 0 0]  TranslationMethod=Cartesian  TranslationCartesianOffset=[stl_x stl_y stl_z]  TranslationCartesianOffsetUnits=m  TranslationStandardAxis=+Z  TranslationStandardOffset=0  TranslationStandardOffsetUnits=m  TranslationROffset=0  TranslationROffsetUnits=m  TranslationThetaOffset=0  TranslationThetaOffsetUnits=deg  TranslationZOffset=0  TranslationZOffsetUnits=m
  W : PMIOPort  Side=Right
  connections:
  Geometry/RConn1 -- Transform Geometry/RConn1
  Transform Geometry/LConn1 -- W/RConn1

== system sm_car/World/Scene/Plane Grid/Grid ==
  Mesh Lines x : Subsystem  mask(Rectangular Mesh){mesh_lenx=grid_x, mesh_leny=grid_y, mesh_hx=hole_wy, mesh_hy=hole_ly, mesh_numhx=1, mesh_numhy=grid_num_sq_y, mesh_thickness=grid_z, mesh_rho=7000, mesh_color=grid_clr, mesh_opc=grid_opc}
      mask prompts: mesh_thickness "Thickness (m)"; mesh_rho "Density (kg/m^3)"; mesh_color "Color [RGB]"; mesh_opc "Opacity (0-1)"
      mask help: Rectangular mesh. Define outer dimensions, dimensions of holes, and thickness. R port is at the CG. Thickness defines the distance of the F frame from the B frame along the z-axis.
      mask init:
      | mesh_xsec = Extr_Data_Mesh(mesh_lenx, mesh_leny, mesh_numhx, mesh_numhy, mesh_hx, mesh_hy);
      mask DialogControl Control12 Prompt: Plot Profile
      mask DialogControl Control12 Callback:
      | v = get_param(gcb,'MaskWSVariables');
      | getMaskValue = containers.Map({v.Name}',{v.Value}');
      | evalin('base',...
      |     sprintf('Extr_Data_Mesh(%s,%s,%s,%s,%s,%s,''%s'');',...
      |     num2str(getMaskValue('mesh_lenx')),...
      |     num2str(getMaskValue('mesh_leny')),...
      |     num2str(getMaskValue('mesh_numhx')),...
      |     num2str(getMaskValue('mesh_numhy')),...
      |     num2str(getMaskValue('mesh_hx')),...
      |     num2str(getMaskValue('mesh_hy')),'plot'));
      mask DialogControl Control7 Prompt: X
      mask DialogControl Control8 Prompt: Y
      mask DialogControl Control9 Prompt: Mesh Length (m)
      mask DialogControl Control11 Prompt: Hole Length (m)
      mask DialogControl Control10 Prompt: Number of Holes
      mask Display: image('Mesh_IMAGE.png');
  "Mesh Lines y " : Subsystem  mask(Rectangular Mesh){mesh_lenx=grid_x, mesh_leny=grid_y, mesh_hx=hole_lx, mesh_hy=hole_wx, mesh_numhx=grid_num_sq_x, mesh_numhy=1, mesh_thickness=grid_z, mesh_rho=7000, mesh_color=grid_clr, mesh_opc=grid_opc}
      mask prompts: mesh_thickness "Thickness (m)"; mesh_rho "Density (kg/m^3)"; mesh_color "Color [RGB]"; mesh_opc "Opacity (0-1)"
      mask help: Rectangular mesh. Define outer dimensions, dimensions of holes, and thickness. R port is at the CG. Thickness defines the distance of the F frame from the B frame along the z-axis.
      mask init:
      | mesh_xsec = Extr_Data_Mesh(mesh_lenx, mesh_leny, mesh_numhx, mesh_numhy, mesh_hx, mesh_hy);
      mask DialogControl Control12 Prompt: Plot Profile
      mask DialogControl Control12 Callback:
      | v = get_param(gcb,'MaskWSVariables');
      | getMaskValue = containers.Map({v.Name}',{v.Value}');
      | evalin('base',...
      |     sprintf('Extr_Data_Mesh(%s,%s,%s,%s,%s,%s,''%s'');',...
      |     num2str(getMaskValue('mesh_lenx')),...
      |     num2str(getMaskValue('mesh_leny')),...
      |     num2str(getMaskValue('mesh_numhx')),...
      |     num2str(getMaskValue('mesh_numhy')),...
      |     num2str(getMaskValue('mesh_hx')),...
      |     num2str(getMaskValue('mesh_hy')),'plot'));
      mask DialogControl Control7 Prompt: X
      mask DialogControl Control8 Prompt: Y
      mask DialogControl Control9 Prompt: Mesh Length (m)
      mask DialogControl Control11 Prompt: Hole Length (m)
      mask DialogControl Control10 Prompt: Number of Holes
      mask Display: image('Mesh_IMAGE.png');
  Reference Frame{,1..3} (4 alike) : sm_lib/Frames and Transforms/Reference Frame
  R : PMIOPort  Side=Left
  connections:
  Reference Frame3/RConn1 -- Mesh Lines x/RConn2
  "Mesh Lines y "/LConn1 -- Mesh Lines x/LConn1 -- R/RConn1
  "Mesh Lines y "/RConn1 -- Reference Frame/RConn1
  Reference Frame1/RConn1 -- "Mesh Lines y "/RConn2
  Reference Frame2/RConn1 -- Mesh Lines x/RConn1

== system sm_car/World/Scene/Plane Grid/Ground Plane ==
  Floor : sm_lib/Body Elements/Brick Solid  BrickDimensions=[gp_l, gp_w, gp_h]  BrickDimensionsUnits=m  ExportEntireGeometry=off  InertiaType=CalculateFromGeometry  BasedOnType=Density  Density=1000  DensityUnits=kg/m^3  Mass=1  MassUnits=kg  CenterOfMass=[0 0 0]  CenterOfMassUnits=m  MomentsOfInertia=[1 1 1]  MomentsOfInertiaUnits=kg*m^2  ProductsOfInertia=[0 0 0]  ProductsOfInertiaUnits=kg*m^2  GraphicType=FromGeometry  MarkerShape=Sphere  MarkerSize=10  GraphicVisPropType=SimpleVisualProperties  GraphicDiffuseColor=gp_clr  GraphicOpacity=gp_opc  GraphicSpecularColor=[0.5 0.5 0.5 1.0]  GraphicAmbientColor=[0.15 0.15 0.15 1.0]  GraphicEmissiveColor=[0.0 0.0 0.0 1.0]  GraphicShininess=75  DoExposeReferenceFrame=off  SerializedFrames=<Frames><Frame><Id>Frame1</Id><Value><Name>F</Name><Origin><Source>GeometricFeature</Source><FeatureName>+z surface</FeatureName></Origin><PrimaryAxis><DefinedDirection>+Z</DefinedDirection><Source>ReferenceFrame</Source><SourceDirection>+Z</SourceDirection><FeatureName></FeatureName></PrimaryAxis><SecondaryAxis><DefinedDirection>+X</DefinedDirection><Source>ReferenceFrame</Source><SourceDirection>+X</SourceDirection><FeatureName></FeatureName></SecondaryAxis></Value></Frame></Frames>
  W : PMIOPort  Side=Right
  connections:
  Floor/LConn1 -- W/RConn1

== system sm_car/World/Scene/Skidpad/Circle Inner L ==
  Solid : sm_lib/Body Elements/Extruded Solid  ExtrusionType=General  PolygonNumSides=3  PolygonOuterRadius=1  PolygonOuterRadiusUnits=m  ExportEntireGeometry=off  ExtrusionCrossSection=xy_data_circ  ExtrusionCrossSectionUnits=m  ExportConvexHullGeometry=off  ExtrusionLength=circ_h  ExtrusionLengthUnits=m  InertiaType=CalculateFromGeometry  BasedOnType=Density  Density=1000  DensityUnits=kg/m^3  Mass=1  MassUnits=kg  CenterOfMass=[0 0 0]  CenterOfMassUnits=m  MomentsOfInertia=[1 1 1]  MomentsOfInertiaUnits=kg*m^2  ProductsOfInertia=[1 1 1]  ProductsOfInertiaUnits=kg*m^2  GraphicType=FromGeometry  MarkerShape=Sphere  MarkerSize=10  GraphicVisPropType=SimpleVisualProperties  GraphicDiffuseColor=[1.0 1.0 0.8]  GraphicOpacity=1.0  GraphicSpecularColor=[0.5 0.5 0.5 1.0]  GraphicAmbientColor=[0.15 0.15 0.15 1.0]  GraphicEmissiveColor=[0.0 0.0 0.0 1.0]  GraphicShininess=75  DoExposeReferenceFrame=on  SerializedFrames=<Frames/>
  W : PMIOPort  Side=Right
  connections:
  Solid/RConn1 -- W/RConn1

== system sm_car/World/Scene/Skidpad/Circle Inner R ==
  Solid : sm_lib/Body Elements/Extruded Solid  ExtrusionType=General  PolygonNumSides=3  PolygonOuterRadius=1  PolygonOuterRadiusUnits=m  ExportEntireGeometry=off  ExtrusionCrossSection=xy_data_circ  ExtrusionCrossSectionUnits=m  ExportConvexHullGeometry=off  ExtrusionLength=circ_h  ExtrusionLengthUnits=m  InertiaType=CalculateFromGeometry  BasedOnType=Density  Density=1000  DensityUnits=kg/m^3  Mass=1  MassUnits=kg  CenterOfMass=[0 0 0]  CenterOfMassUnits=m  MomentsOfInertia=[1 1 1]  MomentsOfInertiaUnits=kg*m^2  ProductsOfInertia=[1 1 1]  ProductsOfInertiaUnits=kg*m^2  GraphicType=FromGeometry  MarkerShape=Sphere  MarkerSize=10  GraphicVisPropType=SimpleVisualProperties  GraphicDiffuseColor=[1.0 1.0 0.8]  GraphicOpacity=1.0  GraphicSpecularColor=[0.5 0.5 0.5 1.0]  GraphicAmbientColor=[0.15 0.15 0.15 1.0]  GraphicEmissiveColor=[0.0 0.0 0.0 1.0]  GraphicShininess=75  DoExposeReferenceFrame=on  SerializedFrames=<Frames/>
  W : PMIOPort  Side=Right
  connections:
  Solid/RConn1 -- W/RConn1

== system sm_car/World/Scene/Skidpad/Circle Outer L ==
  Solid : sm_lib/Body Elements/Extruded Solid  ExtrusionType=General  PolygonNumSides=3  PolygonOuterRadius=1  PolygonOuterRadiusUnits=m  ExportEntireGeometry=off  ExtrusionCrossSection=xy_data_circ  ExtrusionCrossSectionUnits=m  ExportConvexHullGeometry=off  ExtrusionLength=circ_h  ExtrusionLengthUnits=m  InertiaType=CalculateFromGeometry  BasedOnType=Density  Density=1000  DensityUnits=kg/m^3  Mass=1  MassUnits=kg  CenterOfMass=[0 0 0]  CenterOfMassUnits=m  MomentsOfInertia=[1 1 1]  MomentsOfInertiaUnits=kg*m^2  ProductsOfInertia=[1 1 1]  ProductsOfInertiaUnits=kg*m^2  GraphicType=FromGeometry  MarkerShape=Sphere  MarkerSize=10  GraphicVisPropType=SimpleVisualProperties  GraphicDiffuseColor=[1.0 1.0 0.8]  GraphicOpacity=1.0  GraphicSpecularColor=[0.5 0.5 0.5 1.0]  GraphicAmbientColor=[0.15 0.15 0.15 1.0]  GraphicEmissiveColor=[0.0 0.0 0.0 1.0]  GraphicShininess=75  DoExposeReferenceFrame=on  SerializedFrames=<Frames/>
  W : PMIOPort  Side=Right
  connections:
  Solid/RConn1 -- W/RConn1
